simulink subsystem "Joystick_Input_To_Swerve_Drive_sub"  (R2026a)
settings: Solver=VariableStepAuto
undefined symbols (not defined in the file): Boost_Trigger_High_Speed, Boost_Trigger_Low_Speed, Field_Translation_Control_Gain, Field_Translation_Speed_Max, Relative_Steering_Error_Angle_Gain, Relative_Steering_Speed_Max, Relative_Translation_Control_Gain, Relative_Translation_Speed_Max, Steering_Mod_Drv_in, Steering_Mod_Drv_out, Steering_Mod_Str_Rel_in, Steering_Mod_Str_Rel_out, Steering_Relative_Gain, Steering_Twist_Gain, Translation_Twist_Gain
libraries: simulink x13, sl_discontinuities x1, Controls_Components_lib x1
settings Model: Creator=ander  LastModifiedBy=ander

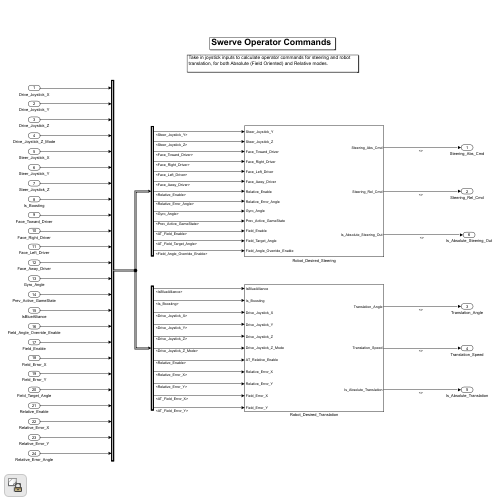
[thumbnail: Simulink's stored preview of the top-level diagram]
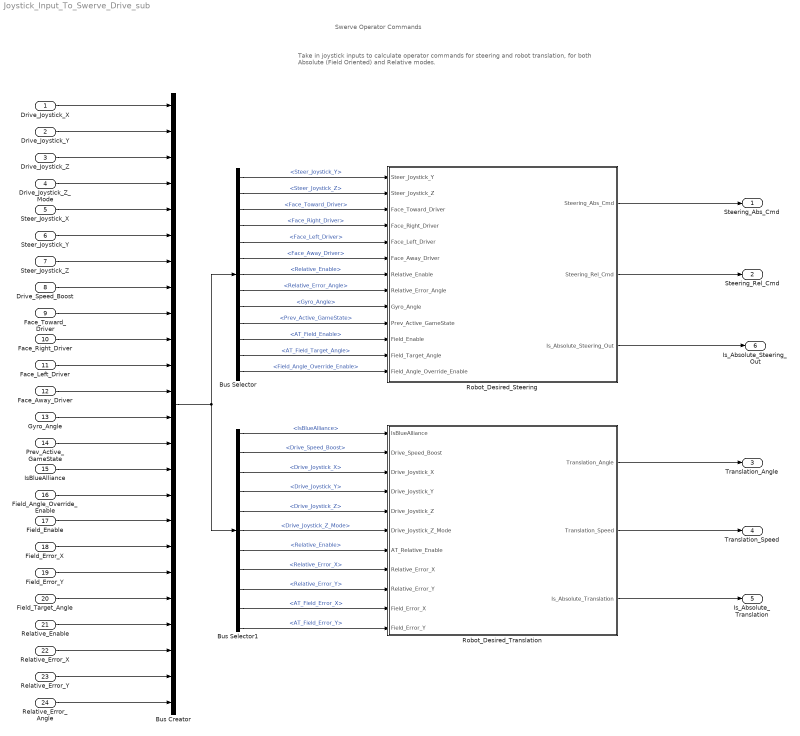
== system Joystick_Input_To_Swerve_Drive_sub ==
  note: Swerve Operator Commands
  note: Take in joystick inputs to calculate operator commands for steering and robot translation, for both Absolute (Field Oriented) and Relative modes.
  Drive_Joystick_X : Inport
  Drive_Joystick_Y : Inport  Port=2
  Drive_Joystick_Z : Inport  Port=3
  Drive_Joystick_Z_Mode : Inport  Port=4
  Steer_Joystick_X : Inport  Port=5
  Steer_Joystick_Y : Inport  Port=6
  Steer_Joystick_Z : Inport  Port=7
  Drive_Speed_Boost : Inport  Port=8
  Face_Toward_Driver : Inport  Port=9
  Face_Right_Driver : Inport  Port=10
  Face_Left_Driver : Inport  Port=11
  Face_Away_Driver : Inport  Port=12
  Gyro_Angle : Inport  Port=13
  Prev_Active_GameState : Inport  Port=14
  IsBlueAlliance : Inport  Port=15
  Field_Angle_Override_Enable : Inport  Port=16
  Field_Enable : Inport  Port=17
  Field_Error_X : Inport  Port=18
  Field_Error_Y : Inport  Port=19
  Field_Target_Angle : Inport  Port=20
  Relative_Enable : Inport  Port=21
  Relative_Error_X : Inport  Port=22
  Relative_Error_Y : Inport  Port=23
  Relative_Error_Angle : Inport  Port=24
  Bus Creator : BusCreator  Inputs=24
  Bus Selector : BusSelector  OutputSignals=Steer_Joystick_Y,Steer_Joystick_Z,Face_Toward_Driver,Face_Right_Driver,Face_Left_Driver,Face_Away_Driver,Relative_Enable,Relative_Error_Angle,Gyro_Angle,Prev_Active_GameState,AT_Field_Enable,AT_Field_Target_Angle,Field_Angle_Override_Enable
  Bus Selector1 : BusSelector  OutputSignals=IsBlueAlliance,Drive_Speed_Boost,Drive_Joystick_X,Drive_Joystick_Y,Drive_Joystick_Z,Drive_Joystick_Z_Mode,Relative_Enable,Relative_Error_X,Relative_Error_Y,AT_Field_Error_X,AT_Field_Error_Y
  Robot_Desired_Steering : Subsystem
  Robot_Desired_Translation : Subsystem
  Steering_Abs_Cmd : Outport
  Steering_Rel_Cmd : Outport  Port=2
  Translation_Angle : Outport  Port=3
  Translation_Speed : Outport  Port=4
  Is_Absolute_Translation : Outport  Port=5
  Is_Absolute_Steering_Out : Outport  Port=6
  wires:
  Relative_Error_Angle/1 -> Bus Creator/24
  Relative_Error_Y/1 -> Bus Creator/23
  Relative_Error_X/1 -> Bus Creator/22
  Relative_Enable/1 -> Bus Creator/21
  Field_Target_Angle/1 -> Bus Creator/20
  Field_Error_Y/1 -> Bus Creator/19
  Field_Error_X/1 -> Bus Creator/18
  Field_Enable/1 -> Bus Creator/17
  Bus Selector1/9 -> Robot_Desired_Translation/9(Relative_Error_Y)  "<Relative_Error_Y>"
  Bus Selector1/8 -> Robot_Desired_Translation/8(Relative_Error_X)  "<Relative_Error_X>"
  Bus Selector1/7 -> Robot_Desired_Translation/7(AT_Relative_Enable)  "<Relative_Enable>"
  Bus Selector/8 -> Robot_Desired_Steering/8(Relative_Error_Angle)  "<Relative_Error_Angle>"
  Robot_Desired_Steering/3(Is_Absolute_Steering_Out) -> Is_Absolute_Steering_Out/1
  Bus Selector1/6 -> Robot_Desired_Translation/6(Drive_Joystick_Z_Mode)  "<Drive_Joystick_Z_Mode>"
  Drive_Joystick_Z_Mode/1 -> Bus Creator/4
  Robot_Desired_Translation/3(Is_Absolute_Translation) -> Is_Absolute_Translation/1
  Bus Selector1/5 -> Robot_Desired_Translation/5(Drive_Joystick_Z)  "<Drive_Joystick_Z>"
  Bus Selector1/2 -> Robot_Desired_Translation/2(Drive_Speed_Boost)  "<Drive_Speed_Boost>"
  Robot_Desired_Steering/2(Steering_Rel_Cmd) -> Steering_Rel_Cmd/1
  Robot_Desired_Steering/1(Steering_Abs_Cmd) -> Steering_Abs_Cmd/1
  Bus Selector/1 -> Robot_Desired_Steering/1(Steer_Joystick_Y)  "<Steer_Joystick_Y>"
  Robot_Desired_Translation/1(Translation_Angle) -> Translation_Angle/1
  Robot_Desired_Translation/2(Translation_Speed) -> Translation_Speed/1
  Bus Creator/1 -> Bus Selector1/1, Bus Selector/1
  Bus Selector1/4 -> Robot_Desired_Translation/4(Drive_Joystick_Y)  "<Drive_Joystick_Y>"
  Bus Selector1/3 -> Robot_Desired_Translation/3(Drive_Joystick_X)  "<Drive_Joystick_X>"
  Drive_Joystick_X/1 -> Bus Creator/1
  Drive_Joystick_Z/1 -> Bus Creator/3
  Steer_Joystick_Y/1 -> Bus Creator/6
  Drive_Joystick_Y/1 -> Bus Creator/2
  Steer_Joystick_X/1 -> Bus Creator/5
  Steer_Joystick_Z/1 -> Bus Creator/7
  Face_Toward_Driver/1 -> Bus Creator/9
  Face_Right_Driver/1 -> Bus Creator/10
  Face_Left_Driver/1 -> Bus Creator/11
  Face_Away_Driver/1 -> Bus Creator/12
  Drive_Speed_Boost/1 -> Bus Creator/8
  Bus Selector/3 -> Robot_Desired_Steering/3(Face_Toward_Driver)  "<Face_Toward_Driver>"
  Bus Selector/2 -> Robot_Desired_Steering/2(Steer_Joystick_Z)  "<Steer_Joystick_Z>"
  Bus Selector/4 -> Robot_Desired_Steering/4(Face_Right_Driver)  "<Face_Right_Driver>"
  Bus Selector/5 -> Robot_Desired_Steering/5(Face_Left_Driver)  "<Face_Left_Driver>"
  Bus Selector/6 -> Robot_Desired_Steering/6(Face_Away_Driver)  "<Face_Away_Driver>"
  Bus Selector1/1 -> Robot_Desired_Translation/1(IsBlueAlliance)  "<IsBlueAlliance>"
  Bus Selector/9 -> Robot_Desired_Steering/9(Gyro_Angle)  "<Gyro_Angle>"
  Bus Selector/7 -> Robot_Desired_Steering/7(Relative_Enable)  "<Relative_Enable>"
  IsBlueAlliance/1 -> Bus Creator/15
  Gyro_Angle/1 -> Bus Creator/13
  Prev_Active_GameState/1 -> Bus Creator/14
  Bus Selector/10 -> Robot_Desired_Steering/10(Prev_Active_GameState)  "<Prev_Active_GameState>"
  Bus Selector/11 -> Robot_Desired_Steering/11(Field_Enable)  "<AT_Field_Enable>"
  Bus Selector/12 -> Robot_Desired_Steering/12(Field_Target_Angle)  "<AT_Field_Target_Angle>"
  Bus Selector1/10 -> Robot_Desired_Translation/10(Field_Error_X)  "<AT_Field_Error_X>"
  Bus Selector1/11 -> Robot_Desired_Translation/11(Field_Error_Y)  "<AT_Field_Error_Y>"
  Field_Angle_Override_Enable/1 -> Bus Creator/16
  Bus Selector/13 -> Robot_Desired_Steering/13(Field_Angle_Override_Enable)  "<Field_Angle_Override_Enable>"

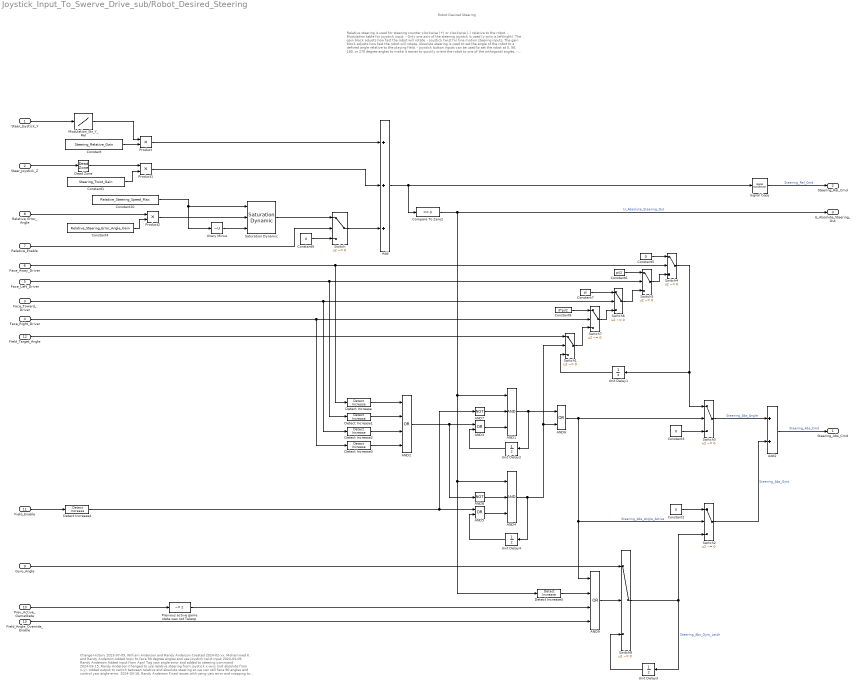
== system Joystick_Input_To_Swerve_Drive_sub/Robot_Desired_Steering ==
  note: Change History
      | 2023-07-09, William Anderson and Randy Anderson
      | Created
      | 2024-02-xx, Mohammed K. and Randy Anderson
      | Added logic to face 90 degree angles and use joystick twist input
      | 2024-03-09, Randy Anderson
      | Added input from April Tag yaw angle error and added to steering command
      | 2024-03-15, Randy Anderson
      | Changed to use relative steering from joystick x-axis (not absolute from x-y).
      | Added output to switch between relative and absolute steering so we can still
      | face 90 angles and control yaw angle error.
      | 2024-03-16, Randy Anderson
      | Fixed issues with using yaw error and snapping to 90 degree angles when
      | coupled with relative steering.
      | 2024-03-18, Randy Anderosn
      | Added gyro angle input to make corrections to robot heading while driving
      | without driver steering input.
      | 2024-03-23, Randy Anderson
      | Changed from April tag yaw error control to April tag angle control.
      | 2024-03-25, Randy Anderson
      | Added twist deadzone.
      | 2025-03-01, Randy Anderson
      | Removed April Tag target angle and replaced with angle error input.
      | Added April Tag enable input.
      | Added maximum relative steering speed for April Tag tracking.
  note: Robot Desired Steering
  note: Relative steering is used for steering counter clockwise (+) or clockwise (-) relative to the robot.
      | - Modulation table for joystick input.
      | - Only one axis of the steering joystck is used (y-axis is left/right). The gain block adjusts how fast the robot will rotate.
      | - Joystick twist for fine motion steering inputs. The gain block adjusts how fast the robot will rotate.
      |
      | Absolute steering is used to set the angle of the robot to a defined angle relative to the playing field.
      | - Joystick button inputs can be used to set the robot at 0, 90, 180, or 270 degree angles to make it easier to quickly orient the robot to one of the orthogonal angles.
      | - April tag target angles are used to set the robot to some input angle corresponding to the location of an April tag. These could be static or dynamic angles. (used in 2024 season, remove in 2025 season)
      | - April tag angle error is an input for relative steering
      | - Gyro angle input is used to compensate for swerve induced robot heading drift while translating. This captures the gyro angle when the relative steering inputs are released and then latches that value as the target heading while there aren't any other active steering commands.
  Steer_Joystick_Y : Inport
  Steer_Joystick_Z : Inport  Port=2
  Face_Toward_Driver : Inport  Port=3
  Face_Right_Driver : Inport  Port=4
  Face_Left_Driver : Inport  Port=5
  Face_Away_Driver : Inport  Port=6
  Relative_Enable : Inport  Port=7
  Relative_Error_Angle : Inport  Port=8
  Gyro_Angle : Inport  Port=9
  Prev_Active_GameState : Inport  Port=10
  Field_Enable : Inport  Port=11
  Field_Target_Angle : Inport  Port=12
  Field_Angle_Override_Enable : Inport  Port=13
  AND1 : Logic  Inputs=3  AllPortsSameDT=off  OutDataTypeStr=boolean
  AND2 : Logic  Operator=OR  Inputs=4  AllPortsSameDT=off  OutDataTypeStr=boolean
  AND3 : Logic  Operator=OR  AllPortsSameDT=off  OutDataTypeStr=boolean
  AND4 : Logic  Inputs=3  AllPortsSameDT=off  OutDataTypeStr=boolean
  AND5 : Logic  Operator=OR  AllPortsSameDT=off  OutDataTypeStr=boolean
  AND6 : Logic  Operator=OR  AllPortsSameDT=off  OutDataTypeStr=boolean
  AND7 : Logic  Operator=NOT  AllPortsSameDT=off  OutDataTypeStr=boolean
  AND8 : Logic  Operator=NOT  AllPortsSameDT=off  OutDataTypeStr=boolean
  AND9 : Logic  Operator=OR  Inputs=4  AllPortsSameDT=off  OutDataTypeStr=boolean
  Add : Sum  Inputs=3
  Add1 : Sum  Inputs=2
  Compare To Zero2 : simulink/Logic and Bit Operations/Compare To Zero  relop===  OutDataTypeStr=boolean
  Constant : Constant  Value=Steering_Relative_Gain
  Constant1 : Constant  Value=Steering_Twist_Gain
  Constant10 : Constant  Value=Relative_Steering_Speed_Max
  Constant{2..3,5,9} (4 alike) : Constant  Value=0
  Constant4 : Constant  Value=Relative_Steering_Error_Angle_Gain
  Constant6 : Constant  Value=pi/2
  Constant7 : Constant  Value=pi
  Constant8 : Constant  Value=3*pi/2
  Dead Zone : DeadZone  LowerValue=Twist_Deadzone_neg  UpperValue=Twist_Deadzone_pos
  Detect Increase{,1..5} (6 alike) : simulink/Logic and Bit Operations/Detect Increase  vinit=0.0  OutDataTypeStr=boolean
  Modulation_Str_Y_Rel : Lookup_n-D  NumberOfTableDimensions=1  BreakpointsForDimension1=Steering_Mod_Str_Rel_in  Table=Steering_Mod_Str_Rel_out  ExtrapMethod=Clip  InternalRulePriority=Speed  RndMeth=Simplest
  Previous active game state was not Teleop : simulink/Logic and Bit Operations/Compare To Constant  relop=~=  const=2  OutDataTypeStr=boolean
  Product : Product
  Product1 : Product
  Product2 : Product
  Saturation Dynamic : sl_discontinuities/Saturation Dynamic  OutMin=[]  OutMax=[]  OutDataTypeStr=Inherit: Same as second input  OutDataType=fixdt(1, 16)  OutScaling=2^-10  DoSatur=off
  Signal Copy : SignalConversion  OverrideOpt=off
  Switch{,1..8} (9 alike) : Switch  Criteria=u2 ~= 0  SaturateOnIntegerOverflow=off  InputSameDT=off
  Unary Minus : UnaryMinus
  Unit Delay{1..4} (4 alike) : UnitDelay  SampleTime=-1
  Steering_Abs_Cmd : Outport
  Steering_Rel_Cmd : Outport  Port=2
  Is_Absolute_Steering_Out : Outport  Port=3
  wires:
  Field_Angle_Override_Enable/1 -> AND9/4
  Unary Minus/1 -> Saturation Dynamic/3
  Constant10/1 -> Saturation Dynamic/1, Unary Minus/1
  Saturation Dynamic/1 -> Switch/1
  Product2/1 -> Saturation Dynamic/2
  Relative_Error_Angle/1 -> Product2/1
  Constant4/1 -> Product2/2
  Field_Target_Angle/1 -> Switch1/1
  Unit Delay1/1 -> Switch1/3
  Switch1/1 -> Switch7/3
  Dead Zone/1 -> Product1/1
  Switch2/1 -> Add1/2  "Steering_Abs_Gyro"
  Constant2/1 -> Switch2/1
  Detect Increase5/1 -> AND9/2
  AND9/1 -> Switch8/2
  AND8/1 -> AND4/2
  AND7/1 -> AND1/2
  AND6/1 -> Switch3/2, AND9/1, Switch2/2  "Steering_Abs_Angle_Active"
  AND4/1 -> AND6/2, Switch1/2, Unit Delay4/1
  Unit Delay4/1 -> AND5/2
  AND5/1 -> AND4/3
  AND2/1 -> AND3/1, AND8/1
  Field_Enable/1 -> Detect Increase4/1
  Detect Increase4/1 -> AND5/1, AND7/1
  Steer_Joystick_Y/1 -> Modulation_Str_Y_Rel/1
  Unit Delay3/1 -> Switch8/3
  Switch8/1 -> Unit Delay3/1, Switch2/3  "Steering_Abs_Gyro_Latch"
  Gyro_Angle/1 -> Switch8/1
  Switch3/1 -> Add1/1  "Steering_Abs_Angle"
  Constant3/1 -> Switch3/3
  Add1/1 -> Steering_Abs_Cmd/1  "Steering_Abs_Cmd"
  Product1/1 -> Add/2
  Product/1 -> Add/1
  Face_Right_Driver/1 -> Detect Increase3/1, Switch7/2
  Face_Toward_Driver/1 -> Detect Increase2/1, Switch6/2
  Face_Left_Driver/1 -> Detect Increase1/1, Switch5/2
  Face_Away_Driver/1 -> Detect Increase/1, Switch4/2
  Switch7/1 -> Switch6/3
  Switch5/1 -> Switch4/3
  Constant8/1 -> Switch7/1
  Constant6/1 -> Switch5/1
  Switch6/1 -> Switch5/3
  Constant7/1 -> Switch6/1
  Constant5/1 -> Switch4/1
  Constant1/1 -> Product1/2
  Steer_Joystick_Z/1 -> Dead Zone/1
  Modulation_Str_Y_Rel/1 -> Product/1
  Add/1 -> Compare To Zero2/1, Signal Copy/1
  Constant/1 -> Product/2
  Switch4/1 -> Switch3/1, Unit Delay1/1
  AND1/1 -> AND6/1, Unit Delay2/1
  Detect Increase/1 -> AND2/1
  Detect Increase1/1 -> AND2/2
  Detect Increase2/1 -> AND2/3
  Detect Increase3/1 -> AND2/4
  AND3/1 -> AND1/3
  Unit Delay2/1 -> AND3/2
  Compare To Zero2/1 -> AND1/1, AND4/1, Detect Increase5/1, Is_Absolute_Steering_Out/1  "Is_Absolute_Steering_Out"
  Signal Copy/1 -> Steering_Rel_Cmd/1  "Steering_Rel_Cmd"
  Prev_Active_GameState/1 -> Previous active game state was not Teleop/1
  Previous active game state was not Teleop/1 -> AND9/3
  Switch/1 -> Add/3
  Relative_Enable/1 -> Switch/2
  Constant9/1 -> Switch/3

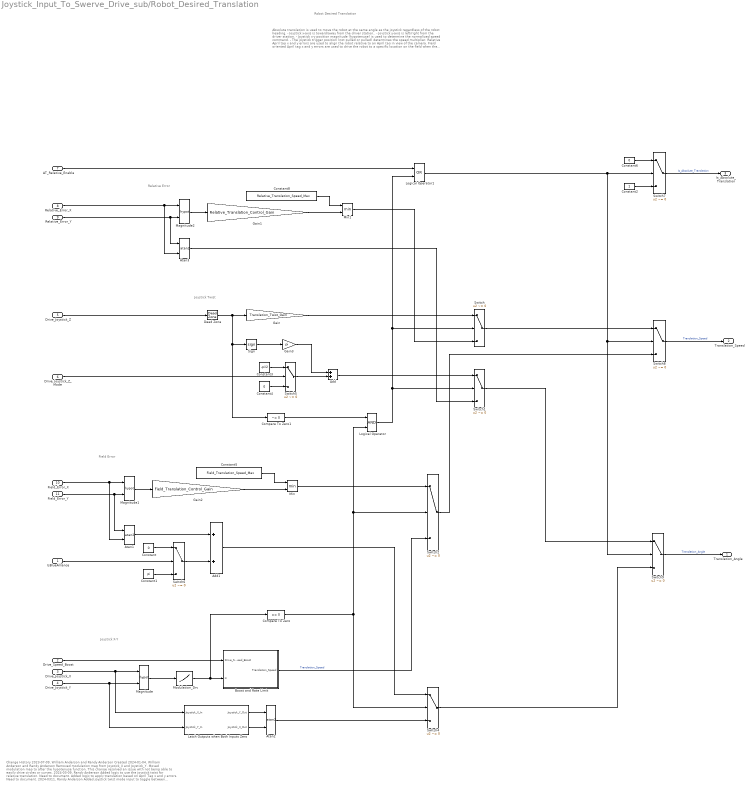
== system Joystick_Input_To_Swerve_Drive_sub/Robot_Desired_Translation ==
  note: Joystick Twist
  note: Relative Error
  note: Change History
      | 2023-07-09, William Anderson and Randy Anderson
      | Created
      | 2024-01-04, William Anderson and Randy Anderson
      | Removed modulation map from Joystick_X and Joystick_Y.
      | Moved modulation map to after the hypotenuse function.
      | This change resolved an issue with not being able to easily drive circles or curves.
      | 2024-03-09, Randy Anderson
      | Added logic to use the joystick twist for relative translation. Need to document.
      | Added logic to apply translation based on April Tag x and y errors. Need to document.
      | 2024-0311, Randy Anderson
      | Added joystick twist mode input to toggle between fwd/rev and left/right relative translation.
      | 2024-03-20, Randy Anderson
      | Changed from IsRedAlliance to IsBlueAlliance and swapped 0 and pi at the switch.
      | 2024-03-25, Randy Anderson
      | Added twist deadzone.
      | 2025-03-01, Randy Anderson
      | Added April Tag enable input.
      | Added maximum relative translation speed for April Tag tracking.
      | 2025-03-03, Randy Anderson
      | Added separate tuning values for relative and field oriented translation speed.
      | Attempted to fix an issue with twist steering (it was only driving forward).
      | Added area blocks to try and separate different modes.
  note: Absolute translation is used to move the robot at the same angle as the joystick regardless of the robot heading.
      | - Joystick x-axis is toward/away from the driver station..
      | - Joystick y-axis is left/right from the driver station.
      | - Joystick x-y position magnitude (hypotenuse) is used to determine the normalized speed command.
      | - The joystick trigger position (not pulled or pulled) determines the speed multiplier.
      |
      | Relative April tag x and y errors are used to align the robot relative to an April tag in view of the camera.
      |
      | Field oriented April tag x and y errors are used to drive the robot to a specific location on the field when the driver has pushed a specific button on the joystick.
      |
      | For both joystick and April tag field oriented steering, use the atan2(y,x) function to determine the absolute heading. The April tag absolute heading needs to be adjusted based on Blue/Red alliance.
      |
      | Relative translation is used to move the robot as if you are driving from the robots prespective.
      | - This is only used when the joystick x-y are centered and there is a joystick z-axis twist.
      | - Twisting will move the robot forward and backward by default.
      | - Twisting will move the robot left and right when another button is also being pushed.
      |
      | The x-y magnitude is passed through a modulation table to provide fine motion control with small inputs.
      | Boost input for increased translation speed.
      | Rate limiter slows down the acceleration of the robot.
      | Angle calculation (atan(y,x)) for absolute translation.
  note: Robot Desired Translation
  note: Field Error
  note: Joystick X-Y
  IsBlueAlliance : Inport
  Drive_Speed_Boost : Inport  Port=2
  Drive_Joystick_X : Inport  Port=3
  Drive_Joystick_Y : Inport  Port=4
  Drive_Joystick_Z : Inport  Port=5
  Drive_Joystick_Z_Mode : Inport  Port=6
  AT_Relative_Enable : Inport  Port=7
  Relative_Error_X : Inport  Port=8
  Relative_Error_Y : Inport  Port=9
  Field_Error_X : Inport  Port=10
  Field_Error_Y : Inport  Port=11
  Add : Sum
  Add1 : Sum
  Atan1 : Trigonometry  Operator=atan2
  Atan2 : Trigonometry  Operator=atan2
  Atan3 : Trigonometry  Operator=atan2
  Boost and Rate Limit : Subsystem
  Compare To Zero : simulink/Logic and Bit Operations/Compare To Zero  relop===  OutDataTypeStr=boolean
  Compare To Zero1 : simulink/Logic and Bit Operations/Compare To Zero  relop=~=  OutDataTypeStr=boolean
  Constant : Constant  Value=0
  Constant1 : Constant  Value=pi
  Constant2 : Constant  OutDataTypeStr=Inherit: Inherit via back propagation
  Constant3 : Constant  Value=-pi/2
  Constant4 : Constant  Value=0
  Constant5 : Constant  Value=Field_Translation_Speed_Max
  Constant6 : Constant  Value=0  OutDataTypeStr=Inherit: Inherit via back propagation
  Constant8 : Constant  Value=Relative_Translation_Speed_Max
  Dead Zone : DeadZone  LowerValue=Twist_Deadzone_neg  UpperValue=Twist_Deadzone_pos
  Gain : Gain  Gain=Translation_Twist_Gain
  Gain1 : Gain  Gain=Relative_Translation_Control_Gain
  Gain2 : Gain  Gain=Field_Translation_Control_Gain
  Gain3 : Gain  Gain=pi
  Latch Outputs when Both Inputs Zero : Subsystem
  Logical Operator : Logic  AllPortsSameDT=off  OutDataTypeStr=boolean
  Logical Operator1 : Logic  Operator=OR  AllPortsSameDT=off  OutDataTypeStr=boolean
  Magnitude : Math  Operator=hypot
  Magnitude1 : Math  Operator=hypot
  Magnitude2 : Math  Operator=hypot
  Min : MinMax  Inputs=2
  Min1 : MinMax  Inputs=2
  Modulation_Drv : Lookup_n-D  NumberOfTableDimensions=1  BreakpointsForDimension1=Steering_Mod_Drv_in  Table=Steering_Mod_Drv_out  ExtrapMethod=Clip  InternalRulePriority=Speed  RndMeth=Simplest
  Sign : Signum
  Switch{,1..2,4..9} (9 alike) : Switch  Criteria=u2 ~= 0  SaturateOnIntegerOverflow=off  InputSameDT=off
  Translation_Angle : Outport
  Translation_Speed : Outport  Port=2
  Is_Absolute_Translation : Outport  Port=3
  wires:
  Gain3/1 -> Add/1
  Add/1 -> Switch1/1
  Sign/1 -> Gain3/1
  Switch5/1 -> Add/2
  Dead Zone/1 -> Gain/1, Sign/1, Compare To Zero1/1
  Atan1/1 -> Add1/1
  Constant/1 -> Switch6/1
  Constant1/1 -> Switch6/3
  Switch6/1 -> Add1/2
  IsBlueAlliance/1 -> Switch6/2
  Add1/1 -> Switch4/1
  Modulation_Drv/1 -> Boost and Rate Limit/2(In), Compare To Zero/1
  Drive_Joystick_Y/1 -> Magnitude/2, Latch Outputs when Both Inputs Zero/2(Joystick_Y_In)
  Drive_Joystick_X/1 -> Magnitude/1, Latch Outputs when Both Inputs Zero/1(Joystick_X_In)
  Magnitude/1 -> Modulation_Drv/1
  Switch9/1 -> Translation_Angle/1  "Translation_Angle"
  Switch8/1 -> Translation_Speed/1  "Translation_Speed"
  Drive_Speed_Boost/1 -> Boost and Rate Limit/1(Drive_Speed_Boost)
  Latch Outputs when Both Inputs Zero/2(Joystick_X_Out) -> Atan2/2
  Latch Outputs when Both Inputs Zero/1(Joystick_Y_Out) -> Atan2/1
  Drive_Joystick_Z/1 -> Dead Zone/1
  Logical Operator/1 -> Logical Operator1/2, Switch/2, Switch1/2
  Compare To Zero1/1 -> Logical Operator/1
  Compare To Zero/1 -> Switch4/2, Switch2/2, Logical Operator/2
  Gain/1 -> Switch/1
  Switch7/1 -> Is_Absolute_Translation/1  "Is_Absolute_Translation"
  Boost and Rate Limit/1(Translation_Speed) -> Switch2/3  "Translation_Speed"
  Field_Error_X/1 -> Atan1/2, Magnitude1/1
  Field_Error_Y/1 -> Magnitude1/2, Atan1/1
  Magnitude1/1 -> Gain2/1
  Atan2/1 -> Switch4/3
  Min/1 -> Switch2/1
  Constant3/1 -> Switch5/1
  Drive_Joystick_Z_Mode/1 -> Switch5/2
  Constant4/1 -> Switch5/3
  Gain2/1 -> Min/2
  Constant5/1 -> Min/1
  Constant6/1 -> Switch7/1
  Constant8/1 -> Min1/1
  Gain1/1 -> Min1/2
  Relative_Error_Y/1 -> Atan3/1, Magnitude2/2
  Relative_Error_X/1 -> Atan3/2, Magnitude2/1
  Magnitude2/1 -> Gain1/1
  Atan3/1 -> Switch1/3
  Min1/1 -> Switch/3
  Constant2/1 -> Switch7/3
  AT_Relative_Enable/1 -> Logical Operator1/1
  Logical Operator1/1 -> Switch9/2, Switch8/2, Switch7/2
  Switch4/1 -> Switch9/3
  Switch2/1 -> Switch8/3
  Switch/1 -> Switch8/1
  Switch1/1 -> Switch9/1

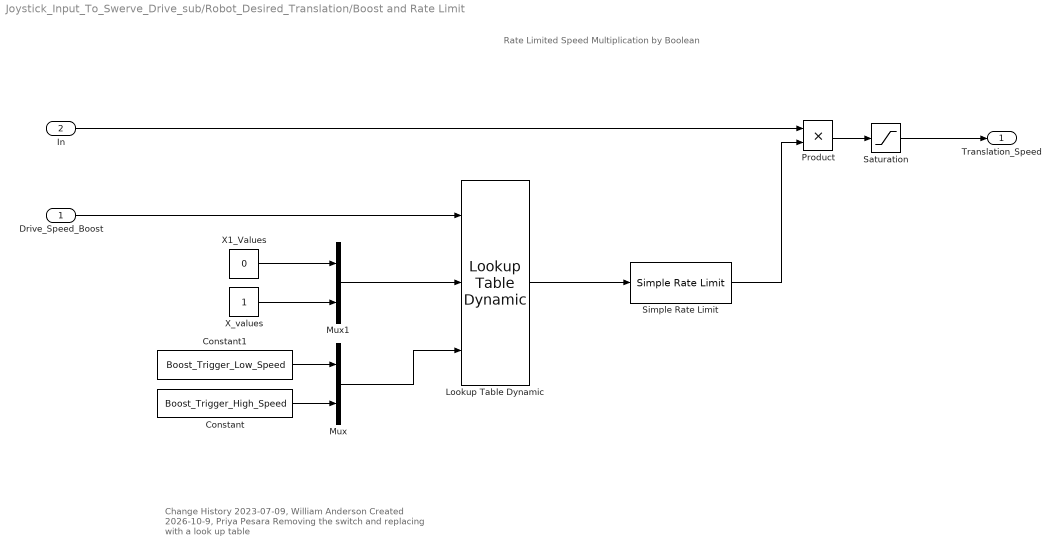
== system Joystick_Input_To_Swerve_Drive_sub/Robot_Desired_Translation/Boost and Rate Limit ==
  note: Change History
      | 2023-07-09, William Anderson
      | Created
      | 2026-10-9, Priya Pesara
      | Removing the switch and replacing with a look up table
  note: Rate Limited Speed Multiplication by Boolean
  Drive_Speed_Boost : Inport
  In : Inport  Port=2
  Constant : Constant  Value=Boost_Trigger_High_Speed
  Constant1 : Constant  Value=Boost_Trigger_Low_Speed
  Lookup Table Dynamic : simulink/Lookup Tables/Lookup Table Dynamic  LookUpMeth=Interpolation-Use End Values  OutDataType=fixdt('double')  OutScaling=[]  OutputDataTypeScalingMode=Specify via dialog  OutDataTypeStr=double  DoSatur=off
  Mux : Mux  Inputs=2
  Mux1 : Mux  Inputs=2
  Product : Product
  Saturation : Saturate  UpperLimit=Boost_Trigger_High_Speed  LowerLimit=-Boost_Trigger_High_Speed
  Simple Rate Limit : Controls_Components_lib/Simple Rate Limit  Rate_Limit_Inc=Boost_Trigger_Increasing_Limit  Rate_Limit_Dec=Boost_Trigger_Decreasing_Limit
  X1_Values : Constant  Value=0
  X_values : Constant
  Translation_Speed : Outport
  wires:
  Constant1/1 -> Mux/1
  Constant/1 -> Mux/2
  Lookup Table Dynamic/1 -> Simple Rate Limit/1
  Mux/1 -> Lookup Table Dynamic/3
  Mux1/1 -> Lookup Table Dynamic/2
  X_values/1 -> Mux1/2
  X1_Values/1 -> Mux1/1
  Drive_Speed_Boost/1 -> Lookup Table Dynamic/1
  In/1 -> Product/1
  Product/1 -> Saturation/1
  Simple Rate Limit/1 -> Product/2
  Saturation/1 -> Translation_Speed/1

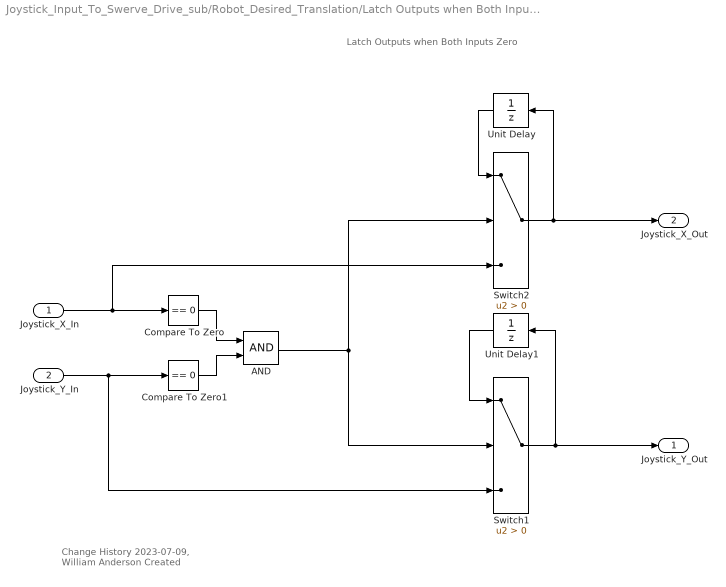
== system Joystick_Input_To_Swerve_Drive_sub/Robot_Desired_Translation/Latch Outputs when Both Inputs Zero ==
  note: Change History
      | 2023-07-09, William Anderson
      | Created
  note: Latch Outputs when Both Inputs Zero
  Joystick_X_In : Inport
  Joystick_Y_In : Inport  Port=2
  AND : Logic  AllPortsSameDT=off  OutDataTypeStr=boolean
  Compare To Zero : simulink/Logic and Bit Operations/Compare To Zero  relop===  OutDataTypeStr=boolean
  Compare To Zero1 : simulink/Logic and Bit Operations/Compare To Zero  relop===  OutDataTypeStr=boolean
  Switch1 : Switch  Criteria=u2 > Threshold  SaturateOnIntegerOverflow=off  InputSameDT=off
  Switch2 : Switch  Criteria=u2 > Threshold  SaturateOnIntegerOverflow=off  InputSameDT=off
  Unit Delay : UnitDelay  SampleTime=-1
  Unit Delay1 : UnitDelay  SampleTime=-1
  Joystick_Y_Out : Outport
  Joystick_X_Out : Outport  Port=2
  wires:
  Switch1/1 -> Joystick_Y_Out/1, Unit Delay1/1
  Switch2/1 -> Joystick_X_Out/1, Unit Delay/1
  Joystick_X_In/1 -> Switch2/3, Compare To Zero/1
  Joystick_Y_In/1 -> Switch1/3, Compare To Zero1/1
  Compare To Zero1/1 -> AND/2
  Compare To Zero/1 -> AND/1
  AND/1 -> Switch1/2, Switch2/2
  Unit Delay/1 -> Switch2/1
  Unit Delay1/1 -> Switch1/1
